simulink model "course_lab5_frequency_second"  (R2024b)
settings: Solver=ode45  StartTime=0.0  StopTime=2.857142857142857  MaxStep=0.001904761904761905  RelTol=1e-7  AbsTol=1e-9
model workspace (MAT data in the model file):
  A = 1
  GBW = 1000000
  K = 1
  T = 0.001
  den = [1 10 500]
  frequency = 3.5
  num = [0 0 500]
  web_input = timeseries
  web_input.Name = 'unnamed'
  web_input.DataInfo = tsdata.datametadata
  web_input.DataInfo.Interpolation = tsdata.interpolation
  web_input.DataInfo.Interpolation.Fhandle : function handle (value not decoded)
  web_input.DataInfo.Interpolation.Name = 'linear'
  web_input.TimeInfo = tsdata.timemetadata
  web_input.TimeInfo.Length = 1501
  web_input.TimeInfo.DuplicateTimes = 0
  web_input.TimeInfo.Time_ = [0 0.00190476190476 0.00380952380952 0.00571428571429 0.00761904761905 0.00952380952381 0.0114285714286 0.0133333333333 0.0152380952381 0.0171428571429 0.0190476190476 0.0209523809524 ... (1501 elements, 1501x1)]
  web_input.TimeInfo.Initialized = 1
  web_input.QualityInfo = tsdata.qualmetadata
  web_input.Data_ = [0 0.0418756537292 0.0836778433323 0.125333233564 0.166768746716 0.207911690818 0.248689887165 0.289031796944 0.328866646739 0.368124552685 0.406736643076 0.444635179185 ... (1501 elements, 1501x1)]
  wn = 22.360679775
  zeta = 0.22360679775
settings Model: Creator=33657  LastModifiedBy=33657

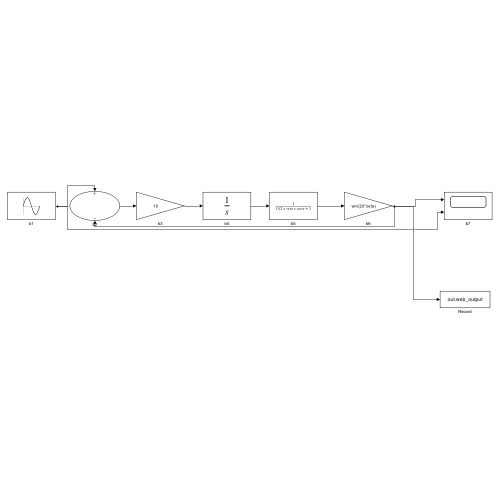
[thumbnail: Simulink's stored preview of the top-level diagram]
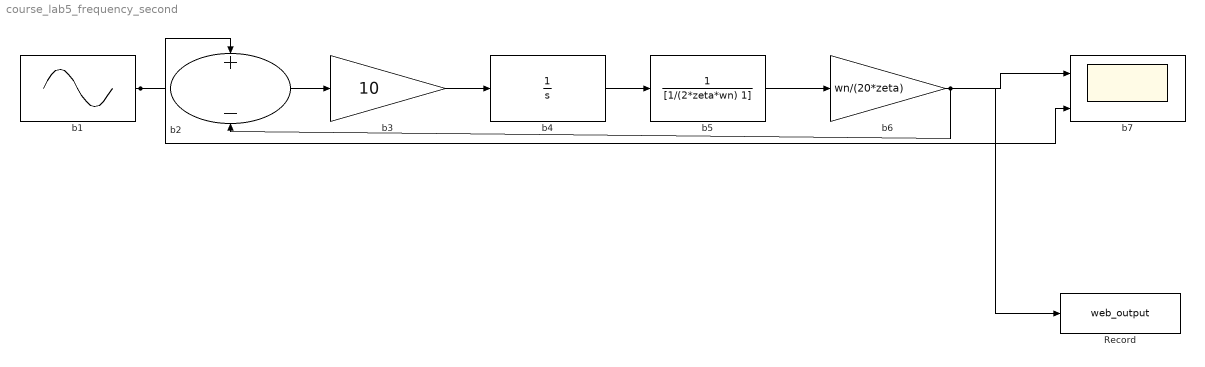
== system course_lab5_frequency_second ==
  Record : ToWorkspace  VariableName=web_output  SaveFormat=Timeseries  SampleTime=-1
  b1 : Sin  Amplitude=A  Frequency=2*pi*frequency  SampleTime=0
  b2 : Sum  Inputs=+-
  b3 : Gain  Gain=10
  b4 : Integrator
  b5 : TransferFcn  Denominator=[1/(2*zeta*wn) 1]
  b6 : Gain  Gain=wn/(20*zeta)
  b7 : Scope  NumInputPorts=2
  wires:
  b1/1 -> b2/1, b7/2
  b2/1 -> b3/1
  b3/1 -> b4/1
  b4/1 -> b5/1
  b5/1 -> b6/1
  b6/1 -> b2/2, b7/1, Record/1
